simulink model "ASM_Traffic_new"  (R2024a)
settings: Solver=ode1  StartTime=SIM.tstart.v  StopTime=SIM.tend.v  FixedStep=SIM.StepSize.v  RelTol=1e-3
PostLoadFcn:
  | if any(exist('dsrtsu_mdlpostloadfcn', 'file') ~= 0), dsrtsu_mdlpostloadfcn('Execute', bdroot); end
  | try, asm_mdl_postloadfcn(bdroot, 'UpdateModel', 3600); catch, disp(lasterr); end,
InitFcn:
  | , if any(exist('rtifpga_mdlclblib', 'file') ~= 0), rtifpga_mdlclblib('Init', bdroot); end,
  | , if any(exist('dsmpb_private', 'file') ~= 0), dsmpb_private('dsmpb_mdlclblib', 'Init', bdroot); end,
undefined symbols (not defined in the file): _to_, a0b2, ASM_BrakeHydraulics_DemoSystems, ASM_VehicleDynamics_DemoSystems, b98103fe8ad365046cd0, BrakeCircuit, CPT, Crankshaft, DiscIntNeverNeededParam, dsmsi, FinalDriveAssembly, MDL, ModeSignals, Pos_BrakePedal_Maneuver, rad, RefSignals, s_to_rpm, SIM, SoftECU, Suspension, Tire, Transmission
libraries: ASM_Traffic_lib x135, simulink x100, ASM_Utils_lib x77, ASM_VehicleDynamics_lib x70, ASM_Environment_lib x22, dsmpblib x20, dsmsilib x15, MDLD_Utils_lib x10, ASM_BrakeHydraulics_lib x3
(part 48 of 63)

== system ASM_Traffic_new/Environment/Sensors/PlantModel/Object_Sensor_3D/ScheduleAndCalculateSensor/GetFellowPositionVector ==
  <FellowPositions> : Inport
  Bus Selector11 : BusSelector  OutputSignals=Pos_Fellows_MainPnt_CoorSys_E[x;y;z][m].Pos_x_Fellows[m],Pos_Fellows_MainPnt_CoorSys_E[x;y;z][m].Pos_y_Fellows[m],Pos_Fellows_MainPnt_CoorSys_E[x;y;z][m].Pos_z_Fellows[m],Angle_Fellows[x;y;z][deg].Angle_Roll_Fellows[deg],Angle_Fellows[x;y;z][deg].Angle_Pitch_Fellows[deg],Angle_Fellows[x;y;z][deg].Angle_Yaw_Fellows[deg]
  Mux1 : Mux  Inputs=3
  Mux2 : Mux  Inputs=3
  Angle_Fellows[deg] : Outport  VectorParamsAs1DForOutWhenUnconnected=off
  Pos_Fellows_MainPnt_CoorSys_E[x;y;z][m] : Outport  Port=2  VectorParamsAs1DForOutWhenUnconnected=off
  wires:
  Mux2/1 -> Pos_Fellows_MainPnt_CoorSys_E[x;y;z][m]/1  "Pos_Fellows_MainPnt_CoorSys_E[x;y;z][m]"
  Mux1/1 -> Angle_Fellows[deg]/1  "Pos_Fellows_MainPnt_CoorSys_E_vec"
  Bus Selector11/4 -> Mux1/1  "<Angle_Roll_Fellows[deg]>"
  Bus Selector11/1 -> Mux2/1  "<Pos_x_Fellows[m]>"
  Bus Selector11/2 -> Mux2/2  "<Pos_y_Fellows[m]>"
  Bus Selector11/6 -> Mux1/3  "<Angle_Yaw_Fellows[deg]>"
  Bus Selector11/5 -> Mux1/2  "<Angle_Pitch_Fellows[deg]>"
  <FellowPositions>/1 -> Bus Selector11/1
  Bus Selector11/3 -> Mux2/3  "<Pos_z_Fellows[m]>"

== system ASM_Traffic_new/Environment/Sensors/PlantModel/Object_Sensor_3D/ScheduleAndCalculateSensor/GetObjectSignals ==
  Traffic_Signals : Inport
  Bus Creator2 : BusCreator  Inputs=3
  Bus Selector3 : BusSelector  OutputSignals=Plant.ObjectParameters.FellowParameters.PosVec_MainPnt_Fellows[x;y;z][m],Plant.ObjectParameters.FellowParameters.Length_Fellows[m],Plant.ObjectParameters.FellowParameters.Width_Fellows[m],Plant.ObjectParameters.FellowParameters.Height_Fellows[m],Plant.ObjectParameters.TrafficObjects.TrafficObject_Type_Data[],Plant.ObjectParameters.FellowParameters.TrafficObject_Type_Fellows[]
  PosVec_MainPnt_Fellows[x;y;z][m] : Outport  VectorParamsAs1DForOutWhenUnconnected=off
  Size_Fellows[m] : Outport  Port=2  VectorParamsAs1DForOutWhenUnconnected=off
  TrafficObject_Type_Data[] : Outport  Port=3  VectorParamsAs1DForOutWhenUnconnected=off
  TrafficObject_Type_Fellows[] : Outport  Port=4  VectorParamsAs1DForOutWhenUnconnected=off
  wires:
  Traffic_Signals/1 -> Bus Selector3/1
  Bus Selector3/2 -> Bus Creator2/1  "<Length_Fellows[m]>"
  Bus Selector3/3 -> Bus Creator2/2  "<Width_Fellows[m]>"
  Bus Selector3/4 -> Bus Creator2/3  "<Height_Fellows[m]>"
  Bus Creator2/1 -> Size_Fellows[m]/1  "Size_Fellows[m]"
  Bus Selector3/1 -> PosVec_MainPnt_Fellows[x;y;z][m]/1  "<PosVec_MainPnt_Fellows[x;y;z][m]>"
  Bus Selector3/5 -> TrafficObject_Type_Data[]/1  "<TrafficObject_Type_Data[]>"
  Bus Selector3/6 -> TrafficObject_Type_Fellows[]/1  "<TrafficObject_Type_Fellows[]>"

== system ASM_Traffic_new/Environment/Sensors/PlantModel/Object_Sensor_3D/ScheduleAndCalculateSensor/SampleAndHold ==
  In1 : Inport
  In2 : Inport  Port=2
  In3 : Inport  Port=3
  In4 : Inport  Port=4
  In5 : Inport  Port=5
  In6 : Inport  Port=6
  In7 : Inport  Port=7
  Enable : EnablePort
  Out1 : Outport  VectorParamsAs1DForOutWhenUnconnected=off
  Out2 : Outport  Port=2  VectorParamsAs1DForOutWhenUnconnected=off
  Out3 : Outport  Port=3  VectorParamsAs1DForOutWhenUnconnected=off
  Out4 : Outport  Port=4  VectorParamsAs1DForOutWhenUnconnected=off
  Out5 : Outport  Port=5  VectorParamsAs1DForOutWhenUnconnected=off
  Out6 : Outport  Port=6  VectorParamsAs1DForOutWhenUnconnected=off
  Out7 : Outport  Port=7  VectorParamsAs1DForOutWhenUnconnected=off
  wires:
  In6/1 -> Out6/1
  In5/1 -> Out5/1
  In4/1 -> Out4/1
  In3/1 -> Out3/1
  In1/1 -> Out1/1
  In2/1 -> Out2/1
  In7/1 -> Out7/1

== system ASM_Traffic_new/Environment/Sensors/PlantModel/Object_Sensor_3D/SensorMapping/Signals_ASMSignalCollector ==
  SensorSignals : Inport
  Bus Creator : BusCreator  Inputs=3
  Bus Selector : BusSelector  OutputSignals=Info.ObjectSensor3D_Sfcn_State[],Info.ObjectSensor3D_Data_Valid[0|1],Info.Flag_Sensor_Init_Ready[0|1]
  Sfcn_Status : Outport  VectorParamsAs1DForOutWhenUnconnected=off
  wires:
  SensorSignals/1 -> Bus Selector/1
  Bus Selector/1 -> Bus Creator/1  "<ObjectSensor3D_Sfcn_State[]>"
  Bus Selector/2 -> Bus Creator/2  "<ObjectSensor3D_Data_Valid[0|1]>"
  Bus Selector/3 -> Bus Creator/3  "<Flag_Sensor_Init_Ready[0|1]>"
  Bus Creator/1 -> Sfcn_Status/1  "Sfcn_Status"

== system ASM_Traffic_new/Environment/Sensors/PlantModel/Object_Sensor_3D/SensorMapping/Signals_to_ACC_SoftECU ==
  Sensor_1_ACC_In : Inport
  Sensor_2_ACC_In : Inport  Port=2
  Bus Creator : BusCreator  Inputs=3
  Bus Creator1 : BusCreator  Inputs=2
  Bus Creator2 : BusCreator  Inputs=4
  Bus Selector : BusSelector  OutputSignals=SensorOutput.Dist_Object[m],SensorOutput.v_Rel_Object[m|s],SensorOutput.Angle_Hor_Object[deg]
  Bus Selector1 : BusSelector  OutputSignals=SensorOutput.Dist_Object[m],SensorOutput.v_Rel_Object[m|s],SensorOutput.Angle_Hor_Object[deg],SensorOutput.Object_ID[]
  Sensor_Signals : Outport  VectorParamsAs1DForOutWhenUnconnected=off
  wires:
  Bus Selector1/3 -> Bus Creator2/3  "<Angle_Hor_Object[deg]>"
  Bus Selector1/2 -> Bus Creator2/2  "<v_Rel_Object[m|s]>"
  Sensor_2_ACC_In/1 -> Bus Selector1/1
  Bus Selector1/4 -> Bus Creator2/4  "<Object_ID[]>"
  Bus Selector1/1 -> Bus Creator2/1  "<Dist_Object[m]>"
  Bus Creator2/1 -> Bus Creator1/2  "Sensor_2_ACC"
  Sensor_1_ACC_In/1 -> Bus Selector/1
  Bus Selector/1 -> Bus Creator/1  "<Dist_Object[m]>"
  Bus Selector/2 -> Bus Creator/2  "<v_Rel_Object[m|s]>"
  Bus Selector/3 -> Bus Creator/3  "<Angle_Hor_Object[deg]>"
  Bus Creator/1 -> Bus Creator1/1  "Sensor_1_ACC"
  Bus Creator1/1 -> Sensor_Signals/1  "SensorSignals"

== system ASM_Traffic_new/Environment/Sensors/PlantModel/Object_Sensor_3D/SensorParameters/ObjectSensor3DParameters_1 ==
  Demux : Demux  Outputs=3
  Demux1 : Demux  Outputs=3
  MODELDESK_GROUP : ASM_Utils_lib/ModelDeskInterface/MODELDESK_GROUP  MDLDGroup=Object Sensor 3D 1  ASMProperties=struct('Name','MODELDESK_GROUP','Version','1.0','Library','ASM_Utils_lib')
  Mux1 : Mux  Inputs=21
  OBJECT_SENSOR_3D_PARAMETERS_1 : ASM_Traffic_lib/Sensors/Object_Sensor_3D/OBJECT_SENSOR_3D_PARAMETERS  Tag=ASM_SUBCOMPONENT  Sw_Sensor_Enable=MDL.Traffic.Sensors.ObjectSensor3D_1.Sw_Sensor_Enable  Const_SensorIdx=MDL.Traffic.Sensors.ObjectSensor3D_1.Const_SensorIdx  Const_t_Offs_Sensor=MDL.Traffic.Sensors.ObjectSensor3D_1.Const_t_Offs_Sensor  Const_t_Cycle_Sensor=MDL.Traffic.Sensors.ObjectSensor3D_1.Const_t_Cycle_Sensor  Const_t_Delay_SensorOutput=MDL.Traffic.Sensors.ObjectSensor3D_1.Const_t_Delay_SensorOutput  Sw_Geometry=MDL.Traffic.Sensors.ObjectSensor3D_1.Sw_Geometry  Const_Pos_Sensor_Apex_CoorSys_V=MDL.Traffic.Sensors.ObjectSensor3D_1.Const_Pos_Sensor_Apex_CoorSys_V  Const_Angle_Orientation_Sensor_CoorSys_V=MDL.Traffic.Sensors.ObjectSensor3D_1.Const_Angle_Orientation_Sensor_CoorSys_V  Const_Length_ScopeZone=MDL.Traffic.Sensors.ObjectSensor3D_1.Const_Length_ScopeZone  Const_Angle_ScopeZone_Horizontal=MDL.Traffic.Sensors.ObjectSensor3D_1.Const_Angle_ScopeZone_Horizontal  Const_Angle_ScopeZone_Vertical=MDL.Traffic.Sensors.ObjectSensor3D_1.Const_Angle_ScopeZone_Vertical  Const_Length_ScopeZone_Head=MDL.Traffic.Sensors.ObjectSensor3D_1.Const_Length_ScopeZone_Head  Const_Length_BlindZone=MDL.Traffic.Sensors.ObjectSensor3D_1.Const_Length_BlindZone  Sw_Occlusion_Mode=MDL.Traffic.Sensors.ObjectSensor3D_1.Sw_Occlusion_Mode  Const_Threshold_Occlusion_Ratio=MDL.Traffic.Sensors.ObjectSensor3D_1.Const_Threshold_Occlusion_Ratio  Sw_Object_Points_Calculation_Enable=MDL.Traffic.Sensors.ObjectSensor3D_1.Sw_Object_Points_Calculation_Enable  Sw_Object_Points_Occlusion_Enable=MDL.Traffic.Sensors.ObjectSensor3D_1.Sw_Object_Points_Occlusion_Enable  ASMProperties=struct('Name','OBJECT_SENSOR_3D_PARAMETERS','Version','4.0','Library','ASM_Traffic_lib')  ASMInstanceName=object_sensor_3d_parameters  ASMInstanceID=1
  Sensor_Parameters[] : Outport  VectorParamsAs1DForOutWhenUnconnected=off
  tag scope: ASMBUS_Environment_Traffic_3DObjSensor1_Parameters=scoped
  wires:
  OBJECT_SENSOR_3D_PARAMETERS_1/18 -> Mux1/21
  OBJECT_SENSOR_3D_PARAMETERS_1/17 -> Mux1/20
  OBJECT_SENSOR_3D_PARAMETERS_1/16 -> Mux1/19
  OBJECT_SENSOR_3D_PARAMETERS_1/15 -> Mux1/18
  Demux1/3 -> Mux1/12
  Demux1/1 -> Mux1/10
  Demux1/2 -> Mux1/11
  Demux/3 -> Mux1/9
  Demux/2 -> Mux1/8
  Demux/1 -> Mux1/7
  OBJECT_SENSOR_3D_PARAMETERS_1/14 -> Mux1/17
  OBJECT_SENSOR_3D_PARAMETERS_1/11 -> Mux1/14
  OBJECT_SENSOR_3D_PARAMETERS_1/6 -> Mux1/5
  OBJECT_SENSOR_3D_PARAMETERS_1/5 -> Mux1/4
  OBJECT_SENSOR_3D_PARAMETERS_1/4 -> Mux1/3
  Mux1/1 -> Sensor_Parameters[]/1
  OBJECT_SENSOR_3D_PARAMETERS_1/10 -> Mux1/13
  OBJECT_SENSOR_3D_PARAMETERS_1/13 -> Mux1/16
  OBJECT_SENSOR_3D_PARAMETERS_1/9 -> Demux1/1
  OBJECT_SENSOR_3D_PARAMETERS_1/8 -> Demux/1
  OBJECT_SENSOR_3D_PARAMETERS_1/1 -> [ASMBUS_Environment_Traffic_3DObjSensor1_Parameters]
  OBJECT_SENSOR_3D_PARAMETERS_1/3 -> Mux1/2
  OBJECT_SENSOR_3D_PARAMETERS_1/2 -> Mux1/1
  OBJECT_SENSOR_3D_PARAMETERS_1/12 -> Mux1/15
  OBJECT_SENSOR_3D_PARAMETERS_1/7 -> Mux1/6

== system ASM_Traffic_new/Environment/Sensors/PlantModel/Object_Sensor_3D/SensorParameters/ObjectSensor3DParameters_2 ==
  Demux2 : Demux  Outputs=3
  Demux3 : Demux  Outputs=3
  MODELDESK_GROUP : ASM_Utils_lib/ModelDeskInterface/MODELDESK_GROUP  MDLDGroup=Object Sensor 3D 2  ASMProperties=struct('Name','MODELDESK_GROUP','Version','1.0','Library','ASM_Utils_lib')
  Mux : Mux  Inputs=21
  OBJECT_SENSOR_3D_PARAMETERS_2 : ASM_Traffic_lib/Sensors/Object_Sensor_3D/OBJECT_SENSOR_3D_PARAMETERS  Tag=ASM_SUBCOMPONENT  Sw_Sensor_Enable=MDL.Traffic.Sensors.ObjectSensor3D_2.Sw_Sensor_Enable  Const_SensorIdx=MDL.Traffic.Sensors.ObjectSensor3D_2.Const_SensorIdx  Const_t_Offs_Sensor=MDL.Traffic.Sensors.ObjectSensor3D_2.Const_t_Offs_Sensor  Const_t_Cycle_Sensor=MDL.Traffic.Sensors.ObjectSensor3D_2.Const_t_Cycle_Sensor  Const_t_Delay_SensorOutput=MDL.Traffic.Sensors.ObjectSensor3D_2.Const_t_Delay_SensorOutput  Sw_Geometry=MDL.Traffic.Sensors.ObjectSensor3D_2.Sw_Geometry  Const_Pos_Sensor_Apex_CoorSys_V=MDL.Traffic.Sensors.ObjectSensor3D_2.Const_Pos_Sensor_Apex_CoorSys_V  Const_Angle_Orientation_Sensor_CoorSys_V=MDL.Traffic.Sensors.ObjectSensor3D_2.Const_Angle_Orientation_Sensor_CoorSys_V  Const_Length_ScopeZone=MDL.Traffic.Sensors.ObjectSensor3D_2.Const_Length_ScopeZone  Const_Angle_ScopeZone_Horizontal=MDL.Traffic.Sensors.ObjectSensor3D_2.Const_Angle_ScopeZone_Horizontal  Const_Angle_ScopeZone_Vertical=MDL.Traffic.Sensors.ObjectSensor3D_2.Const_Angle_ScopeZone_Vertical  Const_Length_ScopeZone_Head=MDL.Traffic.Sensors.ObjectSensor3D_2.Const_Length_ScopeZone_Head  Const_Length_BlindZone=MDL.Traffic.Sensors.ObjectSensor3D_2.Const_Length_BlindZone  Sw_Occlusion_Mode=MDL.Traffic.Sensors.ObjectSensor3D_2.Sw_Occlusion_Mode  Const_Threshold_Occlusion_Ratio=MDL.Traffic.Sensors.ObjectSensor3D_2.Const_Threshold_Occlusion_Ratio  Sw_Object_Points_Calculation_Enable=MDL.Traffic.Sensors.ObjectSensor3D_2.Sw_Object_Points_Calculation_Enable  Sw_Object_Points_Occlusion_Enable=MDL.Traffic.Sensors.ObjectSensor3D_2.Sw_Object_Points_Occlusion_Enable  ASMProperties=struct('Name','OBJECT_SENSOR_3D_PARAMETERS','Version','4.0','Library','ASM_Traffic_lib')  ASMInstanceName=object_sensor_3d_parameters  ASMInstanceID=2
      settings: AttributesFormatString=Instance Name: %<ASMInstanceName>\nInstance ID: %<ASMInstanceID>
  Sensor_Parameters[] : Outport  VectorParamsAs1DForOutWhenUnconnected=off
  tag scope: ASMBUS_Environment_Traffic_3DObjSensor2_Parameters=scoped
  wires:
  OBJECT_SENSOR_3D_PARAMETERS_2/18 -> Mux/21
  OBJECT_SENSOR_3D_PARAMETERS_2/17 -> Mux/20
  OBJECT_SENSOR_3D_PARAMETERS_2/16 -> Mux/19
  OBJECT_SENSOR_3D_PARAMETERS_2/15 -> Mux/18
  Demux3/3 -> Mux/12
  Demux3/1 -> Mux/10
  Demux3/2 -> Mux/11
  Demux2/3 -> Mux/9
  Demux2/1 -> Mux/7
  Demux2/2 -> Mux/8
  Mux/1 -> Sensor_Parameters[]/1
  OBJECT_SENSOR_3D_PARAMETERS_2/14 -> Mux/17
  OBJECT_SENSOR_3D_PARAMETERS_2/12 -> Mux/15
  OBJECT_SENSOR_3D_PARAMETERS_2/1 -> [ASMBUS_Environment_Traffic_3DObjSensor2_Parameters]
  OBJECT_SENSOR_3D_PARAMETERS_2/9 -> Demux3/1
  OBJECT_SENSOR_3D_PARAMETERS_2/10 -> Mux/13
  OBJECT_SENSOR_3D_PARAMETERS_2/3 -> Mux/2
  OBJECT_SENSOR_3D_PARAMETERS_2/7 -> Mux/6
  OBJECT_SENSOR_3D_PARAMETERS_2/4 -> Mux/3
  OBJECT_SENSOR_3D_PARAMETERS_2/13 -> Mux/16
  OBJECT_SENSOR_3D_PARAMETERS_2/8 -> Demux2/1
  OBJECT_SENSOR_3D_PARAMETERS_2/6 -> Mux/5
  OBJECT_SENSOR_3D_PARAMETERS_2/11 -> Mux/14
  OBJECT_SENSOR_3D_PARAMETERS_2/2 -> Mux/1
  OBJECT_SENSOR_3D_PARAMETERS_2/5 -> Mux/4

== system ASM_Traffic_new/Environment/Sensors/PlantModel/Object_Sensor_3D/SensorParameters/ObjectSensor3DParameters_3 ==
  Demux4 : Demux  Outputs=3
  Demux5 : Demux  Outputs=3
  MODELDESK_GROUP : ASM_Utils_lib/ModelDeskInterface/MODELDESK_GROUP  MDLDGroup=Object Sensor 3D 3  ASMProperties=struct('Name','MODELDESK_GROUP','Version','1.0','Library','ASM_Utils_lib')
  Mux2 : Mux  Inputs=21
  OBJECT_SENSOR_3D_PARAMETERS_3 : ASM_Traffic_lib/Sensors/Object_Sensor_3D/OBJECT_SENSOR_3D_PARAMETERS  Tag=ASM_SUBCOMPONENT  Sw_Sensor_Enable=MDL.Traffic.Sensors.ObjectSensor3D_3.Sw_Sensor_Enable  Const_SensorIdx=MDL.Traffic.Sensors.ObjectSensor3D_3.Const_SensorIdx  Const_t_Offs_Sensor=MDL.Traffic.Sensors.ObjectSensor3D_3.Const_t_Offs_Sensor  Const_t_Cycle_Sensor=MDL.Traffic.Sensors.ObjectSensor3D_3.Const_t_Cycle_Sensor  Const_t_Delay_SensorOutput=MDL.Traffic.Sensors.ObjectSensor3D_3.Const_t_Delay_SensorOutput  Sw_Geometry=MDL.Traffic.Sensors.ObjectSensor3D_3.Sw_Geometry  Const_Pos_Sensor_Apex_CoorSys_V=MDL.Traffic.Sensors.ObjectSensor3D_3.Const_Pos_Sensor_Apex_CoorSys_V  Const_Angle_Orientation_Sensor_CoorSys_V=MDL.Traffic.Sensors.ObjectSensor3D_3.Const_Angle_Orientation_Sensor_CoorSys_V  Const_Length_ScopeZone=MDL.Traffic.Sensors.ObjectSensor3D_3.Const_Length_ScopeZone  Const_Angle_ScopeZone_Horizontal=MDL.Traffic.Sensors.ObjectSensor3D_3.Const_Angle_ScopeZone_Horizontal  Const_Angle_ScopeZone_Vertical=MDL.Traffic.Sensors.ObjectSensor3D_3.Const_Angle_ScopeZone_Vertical  Const_Length_ScopeZone_Head=MDL.Traffic.Sensors.ObjectSensor3D_3.Const_Length_ScopeZone_Head  Const_Length_BlindZone=MDL.Traffic.Sensors.ObjectSensor3D_3.Const_Length_BlindZone  Sw_Occlusion_Mode=MDL.Traffic.Sensors.ObjectSensor3D_3.Sw_Occlusion_Mode  Const_Threshold_Occlusion_Ratio=MDL.Traffic.Sensors.ObjectSensor3D_3.Const_Threshold_Occlusion_Ratio  Sw_Object_Points_Calculation_Enable=MDL.Traffic.Sensors.ObjectSensor3D_3.Sw_Object_Points_Calculation_Enable  Sw_Object_Points_Occlusion_Enable=MDL.Traffic.Sensors.ObjectSensor3D_3.Sw_Object_Points_Occlusion_Enable  ASMProperties=struct('Name','OBJECT_SENSOR_3D_PARAMETERS','Version','4.0','Library','ASM_Traffic_lib')  ASMInstanceName=object_sensor_3d_parameters  ASMInstanceID=3
      settings: AttributesFormatString=Instance Name: %<ASMInstanceName>\nInstance ID: %<ASMInstanceID>
  Sensor_Parameters[] : Outport  VectorParamsAs1DForOutWhenUnconnected=off
  tag scope: ASMBUS_Environment_Traffic_3DObjSensor3_Parameters=scoped
  wires:
  OBJECT_SENSOR_3D_PARAMETERS_3/18 -> Mux2/21
  OBJECT_SENSOR_3D_PARAMETERS_3/17 -> Mux2/20
  OBJECT_SENSOR_3D_PARAMETERS_3/16 -> Mux2/19
  OBJECT_SENSOR_3D_PARAMETERS_3/15 -> Mux2/18
  Demux5/3 -> Mux2/9
  Demux5/1 -> Mux2/7
  Demux5/2 -> Mux2/8
  Demux4/3 -> Mux2/12
  Demux4/1 -> Mux2/10
  Demux4/2 -> Mux2/11
  Mux2/1 -> Sensor_Parameters[]/1
  OBJECT_SENSOR_3D_PARAMETERS_3/14 -> Mux2/17
  OBJECT_SENSOR_3D_PARAMETERS_3/13 -> Mux2/16
  OBJECT_SENSOR_3D_PARAMETERS_3/12 -> Mux2/15
  OBJECT_SENSOR_3D_PARAMETERS_3/11 -> Mux2/14
  OBJECT_SENSOR_3D_PARAMETERS_3/10 -> Mux2/13
  OBJECT_SENSOR_3D_PARAMETERS_3/9 -> Demux4/1
  OBJECT_SENSOR_3D_PARAMETERS_3/8 -> Demux5/1
  OBJECT_SENSOR_3D_PARAMETERS_3/7 -> Mux2/6
  OBJECT_SENSOR_3D_PARAMETERS_3/6 -> Mux2/5
  OBJECT_SENSOR_3D_PARAMETERS_3/5 -> Mux2/4
  OBJECT_SENSOR_3D_PARAMETERS_3/4 -> Mux2/3
  OBJECT_SENSOR_3D_PARAMETERS_3/3 -> Mux2/2
  OBJECT_SENSOR_3D_PARAMETERS_3/2 -> Mux2/1
  OBJECT_SENSOR_3D_PARAMETERS_3/1 -> [ASMBUS_Environment_Traffic_3DObjSensor3_Parameters]

== system ASM_Traffic_new/Environment/Sensors/UserInterface/DISP_Plant/Line_Sensor/Data_Valid[0|1|2] ==
  In1 : Inport
  Out1 : Outport  VectorParamsAs1DForOutWhenUnconnected=off
  wires:
  In1/1 -> Out1/1

== system ASM_Traffic_new/Environment/Sensors/UserInterface/DISP_Plant/Line_Sensor/Num_Pnts_Detected_Junction_Borders[] ==
  In1 : Inport
  Out1 : Outport  VectorParamsAs1DForOutWhenUnconnected=off
  wires:
  In1/1 -> Out1/1

== system ASM_Traffic_new/Environment/Sensors/UserInterface/DISP_Plant/Line_Sensor/Num_Pnts_Detected_Junction_Shape_ContObj[] ==
  In1 : Inport
  Out1 : Outport  VectorParamsAs1DForOutWhenUnconnected=off
  wires:
  In1/1 -> Out1/1

== system ASM_Traffic_new/Environment/Sensors/UserInterface/DISP_Plant/Line_Sensor/Num_Pnts_Detected_Junction_Shape_Lines[] ==
  In1 : Inport
  Out1 : Outport  VectorParamsAs1DForOutWhenUnconnected=off
  wires:
  In1/1 -> Out1/1

== system ASM_Traffic_new/Environment/Sensors/UserInterface/DISP_Plant/Line_Sensor/Num_Pnts_Detected_Road_Lanes[] ==
  In1 : Inport
  Out1 : Outport  VectorParamsAs1DForOutWhenUnconnected=off
  wires:
  In1/1 -> Out1/1

== system ASM_Traffic_new/Environment/Sensors/UserInterface/DISP_Plant/Line_Sensor/Num_Pnts_Detected_Road_Shape_ContObj[] ==
  In1 : Inport
  Out1 : Outport  VectorParamsAs1DForOutWhenUnconnected=off
  wires:
  In1/1 -> Out1/1

== system ASM_Traffic_new/Environment/Sensors/UserInterface/DISP_Plant/Line_Sensor/Num_Pnts_Detected_Road_Shape_Lines[] ==
  In1 : Inport
  Out1 : Outport  VectorParamsAs1DForOutWhenUnconnected=off
  wires:
  In1/1 -> Out1/1

== system ASM_Traffic_new/Environment/Sensors/UserInterface/DISP_Plant/Object_Sensor_2D/Angle_Hor_Rel[deg] ==
  In1 : Inport
  Out1 : Outport  VectorParamsAs1DForOutWhenUnconnected=off
  wires:
  In1/1 -> Out1/1

== system ASM_Traffic_new/Environment/Sensors/UserInterface/DISP_Plant/Object_Sensor_2D/Angle_Hor_Rel[deg]1 ==
  In1 : Inport
  Out1 : Outport  VectorParamsAs1DForOutWhenUnconnected=off
  wires:
  In1/1 -> Out1/1

== system ASM_Traffic_new/Environment/Sensors/UserInterface/DISP_Plant/Object_Sensor_2D/Angle_Hor_Rel[deg]2 ==
  In1 : Inport
  Out1 : Outport  VectorParamsAs1DForOutWhenUnconnected=off
  wires:
  In1/1 -> Out1/1

== system ASM_Traffic_new/Environment/Sensors/UserInterface/DISP_Plant/Object_Sensor_2D/Angle_Hor_Rel[deg]3 ==
  In1 : Inport
  Out1 : Outport  VectorParamsAs1DForOutWhenUnconnected=off
  wires:
  In1/1 -> Out1/1

== system ASM_Traffic_new/Environment/Sensors/UserInterface/DISP_Plant/Object_Sensor_2D/Angle_Hor_Rel[deg]4 ==
  In1 : Inport
  Out1 : Outport  VectorParamsAs1DForOutWhenUnconnected=off
  wires:
  In1/1 -> Out1/1

== system ASM_Traffic_new/Environment/Sensors/UserInterface/DISP_Plant/Object_Sensor_2D/Angle_Hor_Rel[deg]5 ==
  In1 : Inport
  Out1 : Outport  VectorParamsAs1DForOutWhenUnconnected=off
  wires:
  In1/1 -> Out1/1

== system ASM_Traffic_new/Environment/Sensors/UserInterface/DISP_Plant/Object_Sensor_2D/Angle_Hor_Rel[deg]6 ==
  In1 : Inport
  Out1 : Outport  VectorParamsAs1DForOutWhenUnconnected=off
  wires:
  In1/1 -> Out1/1

== system ASM_Traffic_new/Environment/Sensors/UserInterface/DISP_Plant/Object_Sensor_2D/Conflict_Flag[0|1] ==
  In1 : Inport
  Out1 : Outport  VectorParamsAs1DForOutWhenUnconnected=off
  wires:
  In1/1 -> Out1/1

== system ASM_Traffic_new/Environment/Sensors/UserInterface/DISP_Plant/Object_Sensor_2D/CycleConflict_Info[] ==
  In1 : Inport
  Out1 : Outport  VectorParamsAs1DForOutWhenUnconnected=off
  wires:
  In1/1 -> Out1/1

== system ASM_Traffic_new/Environment/Sensors/UserInterface/DISP_Plant/Object_Sensor_2D/DelayPulse_SensorOutput[0|1] ==
  In1 : Inport
  Out1 : Outport  VectorParamsAs1DForOutWhenUnconnected=off
  wires:
  In1/1 -> Out1/1

== system ASM_Traffic_new/Environment/Sensors/UserInterface/DISP_Plant/Object_Sensor_2D/Distance[m] ==
  In1 : Inport
  Out1 : Outport  VectorParamsAs1DForOutWhenUnconnected=off
  wires:
  In1/1 -> Out1/1

== system ASM_Traffic_new/Environment/Sensors/UserInterface/DISP_Plant/Object_Sensor_2D/Distance[m]1 ==
  In1 : Inport
  Out1 : Outport  VectorParamsAs1DForOutWhenUnconnected=off
  wires:
  In1/1 -> Out1/1

== system ASM_Traffic_new/Environment/Sensors/UserInterface/DISP_Plant/Object_Sensor_2D/Distance[m]2 ==
  In1 : Inport
  Out1 : Outport  VectorParamsAs1DForOutWhenUnconnected=off
  wires:
  In1/1 -> Out1/1

== system ASM_Traffic_new/Environment/Sensors/UserInterface/DISP_Plant/Object_Sensor_2D/Distance[m]3 ==
  In1 : Inport
  Out1 : Outport  VectorParamsAs1DForOutWhenUnconnected=off
  wires:
  In1/1 -> Out1/1

== system ASM_Traffic_new/Environment/Sensors/UserInterface/DISP_Plant/Object_Sensor_2D/Distance[m]4 ==
  In1 : Inport
  Out1 : Outport  VectorParamsAs1DForOutWhenUnconnected=off
  wires:
  In1/1 -> Out1/1

== system ASM_Traffic_new/Environment/Sensors/UserInterface/DISP_Plant/Object_Sensor_2D/Distance[m]5 ==
  In1 : Inport
  Out1 : Outport  VectorParamsAs1DForOutWhenUnconnected=off
  wires:
  In1/1 -> Out1/1

== system ASM_Traffic_new/Environment/Sensors/UserInterface/DISP_Plant/Object_Sensor_2D/Distance[m]6 ==
  In1 : Inport
  Out1 : Outport  VectorParamsAs1DForOutWhenUnconnected=off
  wires:
  In1/1 -> Out1/1

== system ASM_Traffic_new/Environment/Sensors/UserInterface/DISP_Plant/Object_Sensor_2D/Flag_Object_In_Scope[0Out|1In] ==
  In1 : Inport
  Out1 : Outport  VectorParamsAs1DForOutWhenUnconnected=off
  wires:
  In1/1 -> Out1/1

== system ASM_Traffic_new/Environment/Sensors/UserInterface/DISP_Plant/Object_Sensor_2D/Flag_Object_In_Scope[0Out|1In]1 ==
  In1 : Inport
  Out1 : Outport  VectorParamsAs1DForOutWhenUnconnected=off
  wires:
  In1/1 -> Out1/1

== system ASM_Traffic_new/Environment/Sensors/UserInterface/DISP_Plant/Object_Sensor_2D/Flag_Object_In_Scope[0Out|1In]2 ==
  In1 : Inport
  Out1 : Outport  VectorParamsAs1DForOutWhenUnconnected=off
  wires:
  In1/1 -> Out1/1

== system ASM_Traffic_new/Environment/Sensors/UserInterface/DISP_Plant/Object_Sensor_2D/Flag_Object_In_Scope[0Out|1In]3 ==
  In1 : Inport
  Out1 : Outport  VectorParamsAs1DForOutWhenUnconnected=off
  wires:
  In1/1 -> Out1/1

== system ASM_Traffic_new/Environment/Sensors/UserInterface/DISP_Plant/Object_Sensor_2D/Flag_Object_In_Scope[0Out|1In]4 ==
  In1 : Inport
  Out1 : Outport  VectorParamsAs1DForOutWhenUnconnected=off
  wires:
  In1/1 -> Out1/1

== system ASM_Traffic_new/Environment/Sensors/UserInterface/DISP_Plant/Object_Sensor_2D/Flag_Object_In_Scope[0Out|1In]5 ==
  In1 : Inport
  Out1 : Outport  VectorParamsAs1DForOutWhenUnconnected=off
  wires:
  In1/1 -> Out1/1

== system ASM_Traffic_new/Environment/Sensors/UserInterface/DISP_Plant/Object_Sensor_2D/Flag_Object_In_Scope[0Out|1In]6 ==
  In1 : Inport
  Out1 : Outport  VectorParamsAs1DForOutWhenUnconnected=off
  wires:
  In1/1 -> Out1/1

== system ASM_Traffic_new/Environment/Sensors/UserInterface/DISP_Plant/Object_Sensor_2D/Flag_Sensor_Apex_In_Object[0Out|1In] ==
  In1 : Inport
  Out1 : Outport  VectorParamsAs1DForOutWhenUnconnected=off
  wires:
  In1/1 -> Out1/1

== system ASM_Traffic_new/Environment/Sensors/UserInterface/DISP_Plant/Object_Sensor_2D/Flag_Sensor_Apex_In_Object[0Out|1In]1 ==
  In1 : Inport
  Out1 : Outport  VectorParamsAs1DForOutWhenUnconnected=off
  wires:
  In1/1 -> Out1/1

== system ASM_Traffic_new/Environment/Sensors/UserInterface/DISP_Plant/Object_Sensor_2D/Flag_Sensor_Apex_In_Object[0Out|1In]2 ==
  In1 : Inport
  Out1 : Outport  VectorParamsAs1DForOutWhenUnconnected=off
  wires:
  In1/1 -> Out1/1

== system ASM_Traffic_new/Environment/Sensors/UserInterface/DISP_Plant/Object_Sensor_2D/Flag_Sensor_Apex_In_Object[0Out|1In]3 ==
  In1 : Inport
  Out1 : Outport  VectorParamsAs1DForOutWhenUnconnected=off
  wires:
  In1/1 -> Out1/1

== system ASM_Traffic_new/Environment/Sensors/UserInterface/DISP_Plant/Object_Sensor_2D/Flag_Sensor_Apex_In_Object[0Out|1In]4 ==
  In1 : Inport
  Out1 : Outport  VectorParamsAs1DForOutWhenUnconnected=off
  wires:
  In1/1 -> Out1/1

== system ASM_Traffic_new/Environment/Sensors/UserInterface/DISP_Plant/Object_Sensor_2D/Flag_Sensor_Apex_In_Object[0Out|1In]5 ==
  In1 : Inport
  Out1 : Outport  VectorParamsAs1DForOutWhenUnconnected=off
  wires:
  In1/1 -> Out1/1

== system ASM_Traffic_new/Environment/Sensors/UserInterface/DISP_Plant/Object_Sensor_2D/Flag_Sensor_Apex_In_Object[0Out|1In]6 ==
  In1 : Inport
  Out1 : Outport  VectorParamsAs1DForOutWhenUnconnected=off
  wires:
  In1/1 -> Out1/1

== system ASM_Traffic_new/Environment/Sensors/UserInterface/DISP_Plant/Object_Sensor_2D/GetSensorData_2DSensor_1 ==
  TrafficBus : Inport
  Bus Selector1 : BusSelector  OutputSignals=SensorStatus.Flag_Object_In_Scope[0Out|1In],SensorStatus.Flag_Sensor_Apex_In_Object[0Out|1In],SensorOutput.Angle_Hor_Rel[deg],SensorOutput.Object_ID[],SensorOutput.Object_Type[],SensorOutput.Distance[m],SensorOutput.v_Rel[m|s],SensorOutput.a_Rel[m|s2],SensorOutput.Height_Min[m],SensorOutput.Height_Max[m]
  Flag_Object_In_Scope[0Out|1In] : Outport  VectorParamsAs1DForOutWhenUnconnected=off
  Flag_Sensor_Apex_In_Object[0Out|1In] : Outport  Port=2  VectorParamsAs1DForOutWhenUnconnected=off
  Angle_Hor_Rel[deg] : Outport  Port=3  VectorParamsAs1DForOutWhenUnconnected=off
  Object_ID[] : Outport  Port=4  VectorParamsAs1DForOutWhenUnconnected=off
  Object_Type[] : Outport  Port=5  VectorParamsAs1DForOutWhenUnconnected=off
  Distance[m] : Outport  Port=6  VectorParamsAs1DForOutWhenUnconnected=off
  v_Rel[m|s] : Outport  Port=7  VectorParamsAs1DForOutWhenUnconnected=off
  a_Rel[m|s2] : Outport  Port=8  VectorParamsAs1DForOutWhenUnconnected=off
  Height_Min[m] : Outport  Port=9  VectorParamsAs1DForOutWhenUnconnected=off
  Height_Max[m] : Outport  Port=10  VectorParamsAs1DForOutWhenUnconnected=off
  wires:
  Bus Selector1/2 -> Flag_Sensor_Apex_In_Object[0Out|1In]/1  "<Flag_Sensor_Apex_In_Object[0Out|1In]>"
  Bus Selector1/1 -> Flag_Object_In_Scope[0Out|1In]/1  "<Flag_Object_In_Scope[0Out|1In]>"
  Bus Selector1/10 -> Height_Max[m]/1  "<Height_Max[m]>"
  Bus Selector1/9 -> Height_Min[m]/1  "<Height_Min[m]>"
  Bus Selector1/8 -> a_Rel[m|s2]/1  "<a_Rel[m|s2]>"
  Bus Selector1/7 -> v_Rel[m|s]/1  "<v_Rel[m|s]>"
  Bus Selector1/6 -> Distance[m]/1  "<Distance[m]>"
  Bus Selector1/5 -> Object_Type[]/1  "<Object_Type[]>"
  Bus Selector1/4 -> Object_ID[]/1  "<Object_ID[]>"
  Bus Selector1/3 -> Angle_Hor_Rel[deg]/1  "<Angle_Hor_Rel[deg]>"
  TrafficBus/1 -> Bus Selector1/1

== system ASM_Traffic_new/Environment/Sensors/UserInterface/DISP_Plant/Object_Sensor_2D/GetSensorData_2DSensor_2 ==
  TrafficBus : Inport
  Bus Selector1 : BusSelector  OutputSignals=SensorStatus.Flag_Object_In_Scope[0Out|1In],SensorStatus.Flag_Sensor_Apex_In_Object[0Out|1In],SensorOutput.Angle_Hor_Rel[deg],SensorOutput.Object_ID[],SensorOutput.Object_Type[],SensorOutput.Distance[m],SensorOutput.v_Rel[m|s],SensorOutput.a_Rel[m|s2],SensorOutput.Height_Min[m],SensorOutput.Height_Max[m]
  Flag_Object_In_Scope[0Out|1In] : Outport  VectorParamsAs1DForOutWhenUnconnected=off
  Flag_Sensor_Apex_In_Object[0Out|1In] : Outport  Port=2  VectorParamsAs1DForOutWhenUnconnected=off
  Angle_Hor_Rel[deg] : Outport  Port=3  VectorParamsAs1DForOutWhenUnconnected=off
  Object_ID[] : Outport  Port=4  VectorParamsAs1DForOutWhenUnconnected=off
  Object_Type[] : Outport  Port=5  VectorParamsAs1DForOutWhenUnconnected=off
  Distance[m] : Outport  Port=6  VectorParamsAs1DForOutWhenUnconnected=off
  v_Rel[m|s] : Outport  Port=7  VectorParamsAs1DForOutWhenUnconnected=off
  a_Rel[m|s2] : Outport  Port=8  VectorParamsAs1DForOutWhenUnconnected=off
  Height_Min[m] : Outport  Port=9  VectorParamsAs1DForOutWhenUnconnected=off
  Height_Max[m] : Outport  Port=10  VectorParamsAs1DForOutWhenUnconnected=off
  wires:
  TrafficBus/1 -> Bus Selector1/1
  Bus Selector1/3 -> Angle_Hor_Rel[deg]/1  "<Angle_Hor_Rel[deg]>"
  Bus Selector1/4 -> Object_ID[]/1  "<Object_ID[]>"
  Bus Selector1/5 -> Object_Type[]/1  "<Object_Type[]>"
  Bus Selector1/6 -> Distance[m]/1  "<Distance[m]>"
  Bus Selector1/7 -> v_Rel[m|s]/1  "<v_Rel[m|s]>"
  Bus Selector1/8 -> a_Rel[m|s2]/1  "<a_Rel[m|s2]>"
  Bus Selector1/9 -> Height_Min[m]/1  "<Height_Min[m]>"
  Bus Selector1/10 -> Height_Max[m]/1  "<Height_Max[m]>"
  Bus Selector1/1 -> Flag_Object_In_Scope[0Out|1In]/1  "<Flag_Object_In_Scope[0Out|1In]>"
  Bus Selector1/2 -> Flag_Sensor_Apex_In_Object[0Out|1In]/1  "<Flag_Sensor_Apex_In_Object[0Out|1In]>"

== system ASM_Traffic_new/Environment/Sensors/UserInterface/DISP_Plant/Object_Sensor_2D/GetSensorData_2DSensor_3 ==
  TrafficBus : Inport
  Bus Selector1 : BusSelector  OutputSignals=SensorStatus.Flag_Object_In_Scope[0Out|1In],SensorStatus.Flag_Sensor_Apex_In_Object[0Out|1In],SensorOutput.Angle_Hor_Rel[deg],SensorOutput.Object_ID[],SensorOutput.Object_Type[],SensorOutput.Distance[m],SensorOutput.v_Rel[m|s],SensorOutput.a_Rel[m|s2],SensorOutput.Height_Min[m],SensorOutput.Height_Max[m]
  Flag_Object_In_Scope[0Out|1In] : Outport  VectorParamsAs1DForOutWhenUnconnected=off
  Flag_Sensor_Apex_In_Object[0Out|1In] : Outport  Port=2  VectorParamsAs1DForOutWhenUnconnected=off
  Angle_Hor_Rel[deg] : Outport  Port=3  VectorParamsAs1DForOutWhenUnconnected=off
  Object_ID[] : Outport  Port=4  VectorParamsAs1DForOutWhenUnconnected=off
  Object_Type[] : Outport  Port=5  VectorParamsAs1DForOutWhenUnconnected=off
  Distance[m] : Outport  Port=6  VectorParamsAs1DForOutWhenUnconnected=off
  v_Rel[m|s] : Outport  Port=7  VectorParamsAs1DForOutWhenUnconnected=off
  a_Rel[m|s2] : Outport  Port=8  VectorParamsAs1DForOutWhenUnconnected=off
  Height_Min[m] : Outport  Port=9  VectorParamsAs1DForOutWhenUnconnected=off
  Height_Max[m] : Outport  Port=10  VectorParamsAs1DForOutWhenUnconnected=off
  wires:
  Bus Selector1/2 -> Flag_Sensor_Apex_In_Object[0Out|1In]/1  "<Flag_Sensor_Apex_In_Object[0Out|1In]>"
  Bus Selector1/1 -> Flag_Object_In_Scope[0Out|1In]/1  "<Flag_Object_In_Scope[0Out|1In]>"
  Bus Selector1/10 -> Height_Max[m]/1  "<Height_Max[m]>"
  Bus Selector1/9 -> Height_Min[m]/1  "<Height_Min[m]>"
  Bus Selector1/8 -> a_Rel[m|s2]/1  "<a_Rel[m|s2]>"
  Bus Selector1/7 -> v_Rel[m|s]/1  "<v_Rel[m|s]>"
  Bus Selector1/6 -> Distance[m]/1  "<Distance[m]>"
  Bus Selector1/5 -> Object_Type[]/1  "<Object_Type[]>"
  Bus Selector1/4 -> Object_ID[]/1  "<Object_ID[]>"
  Bus Selector1/3 -> Angle_Hor_Rel[deg]/1  "<Angle_Hor_Rel[deg]>"
  TrafficBus/1 -> Bus Selector1/1

== system ASM_Traffic_new/Environment/Sensors/UserInterface/DISP_Plant/Object_Sensor_2D/GetSensorData_2DSensor_4 ==
  TrafficBus : Inport
  Bus Selector1 : BusSelector  OutputSignals=SensorStatus.Flag_Object_In_Scope[0Out|1In],SensorStatus.Flag_Sensor_Apex_In_Object[0Out|1In],SensorOutput.Angle_Hor_Rel[deg],SensorOutput.Object_ID[],SensorOutput.Object_Type[],SensorOutput.Distance[m],SensorOutput.v_Rel[m|s],SensorOutput.a_Rel[m|s2],SensorOutput.Height_Min[m],SensorOutput.Height_Max[m]
  Flag_Object_In_Scope[0Out|1In] : Outport  VectorParamsAs1DForOutWhenUnconnected=off
  Flag_Sensor_Apex_In_Object[0Out|1In] : Outport  Port=2  VectorParamsAs1DForOutWhenUnconnected=off
  Angle_Hor_Rel[deg] : Outport  Port=3  VectorParamsAs1DForOutWhenUnconnected=off
  Object_ID[] : Outport  Port=4  VectorParamsAs1DForOutWhenUnconnected=off
  Object_Type[] : Outport  Port=5  VectorParamsAs1DForOutWhenUnconnected=off
  Distance[m] : Outport  Port=6  VectorParamsAs1DForOutWhenUnconnected=off
  v_Rel[m|s] : Outport  Port=7  VectorParamsAs1DForOutWhenUnconnected=off
  a_Rel[m|s2] : Outport  Port=8  VectorParamsAs1DForOutWhenUnconnected=off
  Height_Min[m] : Outport  Port=9  VectorParamsAs1DForOutWhenUnconnected=off
  Height_Max[m] : Outport  Port=10  VectorParamsAs1DForOutWhenUnconnected=off
  wires:
  TrafficBus/1 -> Bus Selector1/1
  Bus Selector1/3 -> Angle_Hor_Rel[deg]/1  "<Angle_Hor_Rel[deg]>"
  Bus Selector1/4 -> Object_ID[]/1  "<Object_ID[]>"
  Bus Selector1/5 -> Object_Type[]/1  "<Object_Type[]>"
  Bus Selector1/6 -> Distance[m]/1  "<Distance[m]>"
  Bus Selector1/7 -> v_Rel[m|s]/1  "<v_Rel[m|s]>"
  Bus Selector1/8 -> a_Rel[m|s2]/1  "<a_Rel[m|s2]>"
  Bus Selector1/9 -> Height_Min[m]/1  "<Height_Min[m]>"
  Bus Selector1/10 -> Height_Max[m]/1  "<Height_Max[m]>"
  Bus Selector1/1 -> Flag_Object_In_Scope[0Out|1In]/1  "<Flag_Object_In_Scope[0Out|1In]>"
  Bus Selector1/2 -> Flag_Sensor_Apex_In_Object[0Out|1In]/1  "<Flag_Sensor_Apex_In_Object[0Out|1In]>"

== system ASM_Traffic_new/Environment/Sensors/UserInterface/DISP_Plant/Object_Sensor_2D/GetSensorData_2DSensor_5 ==
  TrafficBus : Inport
  Bus Selector1 : BusSelector  OutputSignals=SensorStatus.Flag_Object_In_Scope[0Out|1In],SensorStatus.Flag_Sensor_Apex_In_Object[0Out|1In],SensorOutput.Angle_Hor_Rel[deg],SensorOutput.Object_ID[],SensorOutput.Object_Type[],SensorOutput.Distance[m],SensorOutput.v_Rel[m|s],SensorOutput.a_Rel[m|s2],SensorOutput.Height_Min[m],SensorOutput.Height_Max[m]
  Flag_Object_In_Scope[0Out|1In] : Outport  VectorParamsAs1DForOutWhenUnconnected=off
  Flag_Sensor_Apex_In_Object[0Out|1In] : Outport  Port=2  VectorParamsAs1DForOutWhenUnconnected=off
  Angle_Hor_Rel[deg] : Outport  Port=3  VectorParamsAs1DForOutWhenUnconnected=off
  Object_ID[] : Outport  Port=4  VectorParamsAs1DForOutWhenUnconnected=off
  Object_Type[] : Outport  Port=5  VectorParamsAs1DForOutWhenUnconnected=off
  Distance[m] : Outport  Port=6  VectorParamsAs1DForOutWhenUnconnected=off
  v_Rel[m|s] : Outport  Port=7  VectorParamsAs1DForOutWhenUnconnected=off
  a_Rel[m|s2] : Outport  Port=8  VectorParamsAs1DForOutWhenUnconnected=off
  Height_Min[m] : Outport  Port=9  VectorParamsAs1DForOutWhenUnconnected=off
  Height_Max[m] : Outport  Port=10  VectorParamsAs1DForOutWhenUnconnected=off
  wires:
  Bus Selector1/2 -> Flag_Sensor_Apex_In_Object[0Out|1In]/1  "<Flag_Sensor_Apex_In_Object[0Out|1In]>"
  Bus Selector1/1 -> Flag_Object_In_Scope[0Out|1In]/1  "<Flag_Object_In_Scope[0Out|1In]>"
  Bus Selector1/10 -> Height_Max[m]/1  "<Height_Max[m]>"
  Bus Selector1/9 -> Height_Min[m]/1  "<Height_Min[m]>"
  Bus Selector1/8 -> a_Rel[m|s2]/1  "<a_Rel[m|s2]>"
  Bus Selector1/7 -> v_Rel[m|s]/1  "<v_Rel[m|s]>"
  Bus Selector1/6 -> Distance[m]/1  "<Distance[m]>"
  Bus Selector1/5 -> Object_Type[]/1  "<Object_Type[]>"
  Bus Selector1/4 -> Object_ID[]/1  "<Object_ID[]>"
  Bus Selector1/3 -> Angle_Hor_Rel[deg]/1  "<Angle_Hor_Rel[deg]>"
  TrafficBus/1 -> Bus Selector1/1

== system ASM_Traffic_new/Environment/Sensors/UserInterface/DISP_Plant/Object_Sensor_2D/GetSensorData_2DSensor_6 ==
  TrafficBus : Inport
  Bus Selector1 : BusSelector  OutputSignals=SensorStatus.Flag_Object_In_Scope[0Out|1In],SensorStatus.Flag_Sensor_Apex_In_Object[0Out|1In],SensorOutput.Angle_Hor_Rel[deg],SensorOutput.Object_ID[],SensorOutput.Object_Type[],SensorOutput.Distance[m],SensorOutput.v_Rel[m|s],SensorOutput.a_Rel[m|s2],SensorOutput.Height_Min[m],SensorOutput.Height_Max[m]
  Flag_Object_In_Scope[0Out|1In] : Outport  VectorParamsAs1DForOutWhenUnconnected=off
  Flag_Sensor_Apex_In_Object[0Out|1In] : Outport  Port=2  VectorParamsAs1DForOutWhenUnconnected=off
  Angle_Hor_Rel[deg] : Outport  Port=3  VectorParamsAs1DForOutWhenUnconnected=off
  Object_ID[] : Outport  Port=4  VectorParamsAs1DForOutWhenUnconnected=off
  Object_Type[] : Outport  Port=5  VectorParamsAs1DForOutWhenUnconnected=off
  Distance[m] : Outport  Port=6  VectorParamsAs1DForOutWhenUnconnected=off
  v_Rel[m|s] : Outport  Port=7  VectorParamsAs1DForOutWhenUnconnected=off
  a_Rel[m|s2] : Outport  Port=8  VectorParamsAs1DForOutWhenUnconnected=off
  Height_Min[m] : Outport  Port=9  VectorParamsAs1DForOutWhenUnconnected=off
  Height_Max[m] : Outport  Port=10  VectorParamsAs1DForOutWhenUnconnected=off
  wires:
  TrafficBus/1 -> Bus Selector1/1
  Bus Selector1/3 -> Angle_Hor_Rel[deg]/1  "<Angle_Hor_Rel[deg]>"
  Bus Selector1/4 -> Object_ID[]/1  "<Object_ID[]>"
  Bus Selector1/5 -> Object_Type[]/1  "<Object_Type[]>"
  Bus Selector1/6 -> Distance[m]/1  "<Distance[m]>"
  Bus Selector1/7 -> v_Rel[m|s]/1  "<v_Rel[m|s]>"
  Bus Selector1/8 -> a_Rel[m|s2]/1  "<a_Rel[m|s2]>"
  Bus Selector1/9 -> Height_Min[m]/1  "<Height_Min[m]>"
  Bus Selector1/10 -> Height_Max[m]/1  "<Height_Max[m]>"
  Bus Selector1/1 -> Flag_Object_In_Scope[0Out|1In]/1  "<Flag_Object_In_Scope[0Out|1In]>"
  Bus Selector1/2 -> Flag_Sensor_Apex_In_Object[0Out|1In]/1  "<Flag_Sensor_Apex_In_Object[0Out|1In]>"

== system ASM_Traffic_new/Environment/Sensors/UserInterface/DISP_Plant/Object_Sensor_2D/GetSensorData_2DSensor_7 ==
  TrafficBus : Inport
  Bus Selector1 : BusSelector  OutputSignals=SensorStatus.Flag_Object_In_Scope[0Out|1In],SensorStatus.Flag_Sensor_Apex_In_Object[0Out|1In],SensorOutput.Angle_Hor_Rel[deg],SensorOutput.Object_ID[],SensorOutput.Object_Type[],SensorOutput.Distance[m],SensorOutput.v_Rel[m|s],SensorOutput.a_Rel[m|s2],SensorOutput.Height_Min[m],SensorOutput.Height_Max[m]
  Flag_Object_In_Scope[0Out|1In] : Outport  VectorParamsAs1DForOutWhenUnconnected=off
  Flag_Sensor_Apex_In_Object[0Out|1In] : Outport  Port=2  VectorParamsAs1DForOutWhenUnconnected=off
  Angle_Hor_Rel[deg] : Outport  Port=3  VectorParamsAs1DForOutWhenUnconnected=off
  Object_ID[] : Outport  Port=4  VectorParamsAs1DForOutWhenUnconnected=off
  Object_Type[] : Outport  Port=5  VectorParamsAs1DForOutWhenUnconnected=off
  Distance[m] : Outport  Port=6  VectorParamsAs1DForOutWhenUnconnected=off
  v_Rel[m|s] : Outport  Port=7  VectorParamsAs1DForOutWhenUnconnected=off
  a_Rel[m|s2] : Outport  Port=8  VectorParamsAs1DForOutWhenUnconnected=off
  Height_Min[m] : Outport  Port=9  VectorParamsAs1DForOutWhenUnconnected=off
  Height_Max[m] : Outport  Port=10  VectorParamsAs1DForOutWhenUnconnected=off
  wires:
  Bus Selector1/2 -> Flag_Sensor_Apex_In_Object[0Out|1In]/1  "<Flag_Sensor_Apex_In_Object[0Out|1In]>"
  Bus Selector1/1 -> Flag_Object_In_Scope[0Out|1In]/1  "<Flag_Object_In_Scope[0Out|1In]>"
  Bus Selector1/10 -> Height_Max[m]/1  "<Height_Max[m]>"
  Bus Selector1/9 -> Height_Min[m]/1  "<Height_Min[m]>"
  Bus Selector1/8 -> a_Rel[m|s2]/1  "<a_Rel[m|s2]>"
  Bus Selector1/7 -> v_Rel[m|s]/1  "<v_Rel[m|s]>"
  Bus Selector1/6 -> Distance[m]/1  "<Distance[m]>"
  Bus Selector1/5 -> Object_Type[]/1  "<Object_Type[]>"
  Bus Selector1/4 -> Object_ID[]/1  "<Object_ID[]>"
  Bus Selector1/3 -> Angle_Hor_Rel[deg]/1  "<Angle_Hor_Rel[deg]>"
  TrafficBus/1 -> Bus Selector1/1

== system ASM_Traffic_new/Environment/Sensors/UserInterface/DISP_Plant/Object_Sensor_2D/Height_Max[m] ==
  In1 : Inport
  Out1 : Outport  VectorParamsAs1DForOutWhenUnconnected=off
  wires:
  In1/1 -> Out1/1

== system ASM_Traffic_new/Environment/Sensors/UserInterface/DISP_Plant/Object_Sensor_2D/Height_Max[m]1 ==
  In1 : Inport
  Out1 : Outport  VectorParamsAs1DForOutWhenUnconnected=off
  wires:
  In1/1 -> Out1/1

== system ASM_Traffic_new/Environment/Sensors/UserInterface/DISP_Plant/Object_Sensor_2D/Height_Max[m]2 ==
  In1 : Inport
  Out1 : Outport  VectorParamsAs1DForOutWhenUnconnected=off
  wires:
  In1/1 -> Out1/1

== system ASM_Traffic_new/Environment/Sensors/UserInterface/DISP_Plant/Object_Sensor_2D/Height_Max[m]3 ==
  In1 : Inport
  Out1 : Outport  VectorParamsAs1DForOutWhenUnconnected=off
  wires:
  In1/1 -> Out1/1

== system ASM_Traffic_new/Environment/Sensors/UserInterface/DISP_Plant/Object_Sensor_2D/Height_Max[m]4 ==
  In1 : Inport
  Out1 : Outport  VectorParamsAs1DForOutWhenUnconnected=off
  wires:
  In1/1 -> Out1/1

== system ASM_Traffic_new/Environment/Sensors/UserInterface/DISP_Plant/Object_Sensor_2D/Height_Max[m]5 ==
  In1 : Inport
  Out1 : Outport  VectorParamsAs1DForOutWhenUnconnected=off
  wires:
  In1/1 -> Out1/1

== system ASM_Traffic_new/Environment/Sensors/UserInterface/DISP_Plant/Object_Sensor_2D/Height_Max[m]6 ==
  In1 : Inport
  Out1 : Outport  VectorParamsAs1DForOutWhenUnconnected=off
  wires:
  In1/1 -> Out1/1

== system ASM_Traffic_new/Environment/Sensors/UserInterface/DISP_Plant/Object_Sensor_2D/Height_Min[m] ==
  In1 : Inport
  Out1 : Outport  VectorParamsAs1DForOutWhenUnconnected=off
  wires:
  In1/1 -> Out1/1

== system ASM_Traffic_new/Environment/Sensors/UserInterface/DISP_Plant/Object_Sensor_2D/Height_Min[m]1 ==
  In1 : Inport
  Out1 : Outport  VectorParamsAs1DForOutWhenUnconnected=off
  wires:
  In1/1 -> Out1/1

== system ASM_Traffic_new/Environment/Sensors/UserInterface/DISP_Plant/Object_Sensor_2D/Height_Min[m]2 ==
  In1 : Inport
  Out1 : Outport  VectorParamsAs1DForOutWhenUnconnected=off
  wires:
  In1/1 -> Out1/1

== system ASM_Traffic_new/Environment/Sensors/UserInterface/DISP_Plant/Object_Sensor_2D/Height_Min[m]3 ==
  In1 : Inport
  Out1 : Outport  VectorParamsAs1DForOutWhenUnconnected=off
  wires:
  In1/1 -> Out1/1

== system ASM_Traffic_new/Environment/Sensors/UserInterface/DISP_Plant/Object_Sensor_2D/Height_Min[m]4 ==
  In1 : Inport
  Out1 : Outport  VectorParamsAs1DForOutWhenUnconnected=off
  wires:
  In1/1 -> Out1/1

== system ASM_Traffic_new/Environment/Sensors/UserInterface/DISP_Plant/Object_Sensor_2D/Height_Min[m]5 ==
  In1 : Inport
  Out1 : Outport  VectorParamsAs1DForOutWhenUnconnected=off
  wires:
  In1/1 -> Out1/1

== system ASM_Traffic_new/Environment/Sensors/UserInterface/DISP_Plant/Object_Sensor_2D/Height_Min[m]6 ==
  In1 : Inport
  Out1 : Outport  VectorParamsAs1DForOutWhenUnconnected=off
  wires:
  In1/1 -> Out1/1

== system ASM_Traffic_new/Environment/Sensors/UserInterface/DISP_Plant/Object_Sensor_2D/IdxSelect_2DSensor ==
  Sensor_1 : Inport
  Sensor_2 : Inport  Port=2
  Sensor_3 : Inport  Port=3
  Sensor_4 : Inport  Port=4
  Sensor_5 : Inport  Port=5
  Sensor_6 : Inport  Port=6
  Sensor_7 : Inport  Port=7
  Bus Selector2 : BusSelector  OutputSignals=SensorStatus.Flag_Object_In_Scope[0Out|1In],SensorStatus.Flag_Sensor_Apex_In_Object[0Out|1In],SensorOutput.Angle_Hor_Rel[deg],SensorOutput.Object_ID[],SensorOutput.Object_Type[],SensorOutput.Distance[m],SensorOutput.v_Rel[m|s],SensorOutput.a_Rel[m|s2],SensorOutput.Height_Min[m],SensorOutput.Height_Max[m]
  Const_Scopezon_El_Idx_1[1_60] : Constant
  Const_Scopezon_El_Idx_2[1_60] : Constant  Value=2
  Const_Scopezon_El_Idx_3[1_60] : Constant  Value=3
  Const_Scopezon_El_Idx_4[1_60] : Constant  Value=4
  Const_Scopezon_El_Idx_5[1_60] : Constant  Value=5
  Multiport Switch : MultiPortSwitch  Inputs=7  SaturateOnIntegerOverflow=off  InputSameDT=off
  Scopezone_Element_Data_Selection1 : Subsystem
  Scopezone_Element_Data_Selection2 : Subsystem
  Scopezone_Element_Data_Selection3 : Subsystem
  Scopezone_Element_Data_Selection4 : Subsystem
  Scopezone_Element_Data_Selection5 : Subsystem
  Sw_Sensor_Selector[] : Constant
  wires:
  Const_Scopezon_El_Idx_5[1_60]/1 -> Scopezone_Element_Data_Selection5/1(Scopezone_El_Idx[1_60])
  Const_Scopezon_El_Idx_4[1_60]/1 -> Scopezone_Element_Data_Selection4/1(Scopezone_El_Idx[1_60])
  Const_Scopezon_El_Idx_3[1_60]/1 -> Scopezone_Element_Data_Selection3/1(Scopezone_El_Idx[1_60])
  Const_Scopezon_El_Idx_2[1_60]/1 -> Scopezone_Element_Data_Selection2/1(Scopezone_El_Idx[1_60])
  Const_Scopezon_El_Idx_1[1_60]/1 -> Scopezone_Element_Data_Selection1/1(Scopezone_El_Idx[1_60])
  Multiport Switch/1 -> Bus Selector2/1
  Bus Selector2/3 -> Scopezone_Element_Data_Selection1/4(Angle_Hor_Rel[deg]), Scopezone_Element_Data_Selection4/4(Angle_Hor_Rel[deg]), Scopezone_Element_Data_Selection5/4(Angle_Hor_Rel[deg]), Scopezone_Element_Data_Selection3/4(Angle_Hor_Rel[deg]), Scopezone_Element_Data_Selection2/4(Angle_Hor_Rel[deg])  "<Angle_Hor_Rel[deg]>"
  Bus Selector2/4 -> Scopezone_Element_Data_Selection4/5(Object_ID[]), Scopezone_Element_Data_Selection5/5(Object_ID[]), Scopezone_Element_Data_Selection3/5(Object_ID[]), Scopezone_Element_Data_Selection2/5(Object_ID[]), Scopezone_Element_Data_Selection1/5(Object_ID[])  "<Object_ID[]>"
  Bus Selector2/5 -> Scopezone_Element_Data_Selection3/6(Object_Type[]), Scopezone_Element_Data_Selection4/6(Object_Type[]), Scopezone_Element_Data_Selection5/6(Object_Type[]), Scopezone_Element_Data_Selection2/6(Object_Type[]), Scopezone_Element_Data_Selection1/6(Object_Type[])  "<Object_Type[]>"
  Bus Selector2/6 -> Scopezone_Element_Data_Selection4/7(Distance[m]), Scopezone_Element_Data_Selection5/7(Distance[m]), Scopezone_Element_Data_Selection3/7(Distance[m]), Scopezone_Element_Data_Selection2/7(Distance[m]), Scopezone_Element_Data_Selection1/7(Distance[m])  "<Distance[m]>"
  Bus Selector2/7 -> Scopezone_Element_Data_Selection4/8(v_Rel[m|s]), Scopezone_Element_Data_Selection5/8(v_Rel[m|s]), Scopezone_Element_Data_Selection3/8(v_Rel[m|s]), Scopezone_Element_Data_Selection2/8(v_Rel[m|s]), Scopezone_Element_Data_Selection1/8(v_Rel[m|s])  "<v_Rel[m|s]>"
  Bus Selector2/8 -> Scopezone_Element_Data_Selection4/9(a_Rel[m|s2]), Scopezone_Element_Data_Selection5/9(a_Rel[m|s2]), Scopezone_Element_Data_Selection3/9(a_Rel[m|s2]), Scopezone_Element_Data_Selection2/9(a_Rel[m|s2]), Scopezone_Element_Data_Selection1/9(a_Rel[m|s2])  "<a_Rel[m|s2]>"
  Bus Selector2/9 -> Scopezone_Element_Data_Selection4/10(Height_Min[m]), Scopezone_Element_Data_Selection5/10(Height_Min[m]), Scopezone_Element_Data_Selection3/10(Height_Min[m]), Scopezone_Element_Data_Selection2/10(Height_Min[m]), Scopezone_Element_Data_Selection1/10(Height_Min[m])  "<Height_Min[m]>"
  Bus Selector2/10 -> Scopezone_Element_Data_Selection4/11(Height_Max[m]), Scopezone_Element_Data_Selection5/11(Height_Max[m]), Scopezone_Element_Data_Selection3/11(Height_Max[m]), Scopezone_Element_Data_Selection2/11(Height_Max[m]), Scopezone_Element_Data_Selection1/11(Height_Max[m])  "<Height_Max[m]>"
  Bus Selector2/1 -> Scopezone_Element_Data_Selection1/2(Flag_Object_In_Scope[0Out|1In]), Scopezone_Element_Data_Selection4/2(Flag_Object_In_Scope[0Out|1In]), Scopezone_Element_Data_Selection5/2(Flag_Object_In_Scope[0Out|1In]), Scopezone_Element_Data_Selection3/2(Flag_Object_In_Scope[0Out|1In]), Scopezone_Element_Data_Selection2/2(Flag_Object_In_Scope[0Out|1In])  "<Flag_Object_In_Scope[0Out|1In]>"
  Bus Selector2/2 -> Scopezone_Element_Data_Selection1/3(Flag_Sensor_Apex_In_Object[0Out|1In]), Scopezone_Element_Data_Selection4/3(Flag_Sensor_Apex_In_Object[0Out|1In]), Scopezone_Element_Data_Selection5/3(Flag_Sensor_Apex_In_Object[0Out|1In]), Scopezone_Element_Data_Selection3/3(Flag_Sensor_Apex_In_Object[0Out|1In]), Scopezone_Element_Data_Selection2/3(Flag_Sensor_Apex_In_Object[0Out|1In])  "<Flag_Sensor_Apex_In_Object[0Out|1In]>"
  Sensor_7/1 -> Multiport Switch/8
  Sensor_6/1 -> Multiport Switch/7
  Sensor_5/1 -> Multiport Switch/6
  Sensor_4/1 -> Multiport Switch/5
  Sw_Sensor_Selector[]/1 -> Multiport Switch/1
  Sensor_1/1 -> Multiport Switch/2
  Sensor_2/1 -> Multiport Switch/3
  Sensor_3/1 -> Multiport Switch/4

== system ASM_Traffic_new/Environment/Sensors/UserInterface/DISP_Plant/Object_Sensor_2D/IndexConflict_Info[] ==
  In1 : Inport
  Out1 : Outport  VectorParamsAs1DForOutWhenUnconnected=off
  wires:
  In1/1 -> Out1/1

== system ASM_Traffic_new/Environment/Sensors/UserInterface/DISP_Plant/Object_Sensor_2D/InputDataSamplePulse[0|1] ==
  In1 : Inport
  Out1 : Outport  VectorParamsAs1DForOutWhenUnconnected=off
  wires:
  In1/1 -> Out1/1

== system ASM_Traffic_new/Environment/Sensors/UserInterface/DISP_Plant/Object_Sensor_2D/ObjectSensor2D_Data_Valid[0|1] ==
  In1 : Inport
  Out1 : Outport  VectorParamsAs1DForOutWhenUnconnected=off
  wires:
  In1/1 -> Out1/1

== system ASM_Traffic_new/Environment/Sensors/UserInterface/DISP_Plant/Object_Sensor_2D/ObjectSensor2D_Sfcn_State[] ==
  In1 : Inport
  Out1 : Outport  VectorParamsAs1DForOutWhenUnconnected=off
  wires:
  In1/1 -> Out1/1

== system ASM_Traffic_new/Environment/Sensors/UserInterface/DISP_Plant/Object_Sensor_2D/Object_ID[] ==
  In1 : Inport
  Out1 : Outport  VectorParamsAs1DForOutWhenUnconnected=off
  wires:
  In1/1 -> Out1/1

== system ASM_Traffic_new/Environment/Sensors/UserInterface/DISP_Plant/Object_Sensor_2D/Object_ID[]1 ==
  In1 : Inport
  Out1 : Outport  VectorParamsAs1DForOutWhenUnconnected=off
  wires:
  In1/1 -> Out1/1

== system ASM_Traffic_new/Environment/Sensors/UserInterface/DISP_Plant/Object_Sensor_2D/Object_ID[]2 ==
  In1 : Inport
  Out1 : Outport  VectorParamsAs1DForOutWhenUnconnected=off
  wires:
  In1/1 -> Out1/1

== system ASM_Traffic_new/Environment/Sensors/UserInterface/DISP_Plant/Object_Sensor_2D/Object_ID[]3 ==
  In1 : Inport
  Out1 : Outport  VectorParamsAs1DForOutWhenUnconnected=off
  wires:
  In1/1 -> Out1/1

== system ASM_Traffic_new/Environment/Sensors/UserInterface/DISP_Plant/Object_Sensor_2D/Object_ID[]4 ==
  In1 : Inport
  Out1 : Outport  VectorParamsAs1DForOutWhenUnconnected=off
  wires:
  In1/1 -> Out1/1

== system ASM_Traffic_new/Environment/Sensors/UserInterface/DISP_Plant/Object_Sensor_2D/Object_ID[]5 ==
  In1 : Inport
  Out1 : Outport  VectorParamsAs1DForOutWhenUnconnected=off
  wires:
  In1/1 -> Out1/1

== system ASM_Traffic_new/Environment/Sensors/UserInterface/DISP_Plant/Object_Sensor_2D/Object_ID[]6 ==
  In1 : Inport
  Out1 : Outport  VectorParamsAs1DForOutWhenUnconnected=off
  wires:
  In1/1 -> Out1/1
